simulink model "EngineInertia"  (R2025b)
settings: Solver=ode1  StartTime=0.0  StopTime=10.0  FixedStep=0.001  RelTol=1e-3
undefined symbols (not defined in the file): omega_e0, Theta_e
settings Model: Creator=williamvandevoir  LastModifiedBy=williamvandevoir

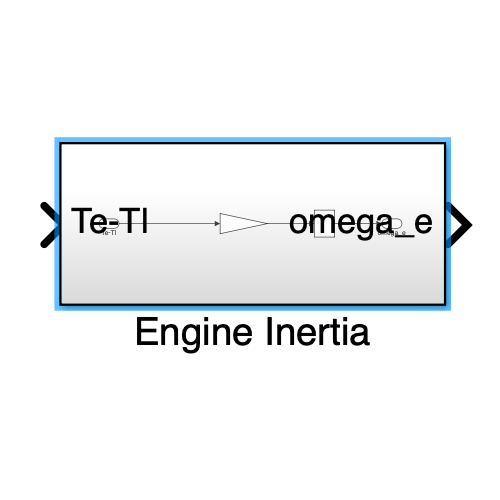
[thumbnail: Simulink's stored preview of the top-level diagram]
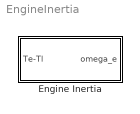
== system EngineInertia ==
  Engine Inertia : Subsystem

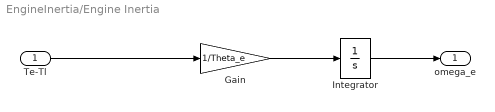
== system EngineInertia/Engine Inertia ==
  Te-Tl : Inport
  Gain : Gain  Gain=1/Theta_e
  Integrator : Integrator  InitialCondition=omega_e0
  omega_e : Outport
  wires:
  Gain/1 -> Integrator/1
  Integrator/1 -> omega_e/1
  Te-Tl/1 -> Gain/1
